simulink model "test_pmsm_inverter"  (R2026b)
settings: Solver=ode23tb  StopTime=tb.t_stop
undefined symbols (not defined in the file or in its folder): mach, tb
libraries: fl_lib x6, nesl_utility x3, permanent_magnet_synchronous_machine x1, pmsm_inverter_dqctrl x1
settings Model: Creator=pwr-control  LastModifiedBy=dbagn
settings SolverCC: ZeroCrossAlgorithm=Adaptive  ZeroCrossControl=EnableAll
settings DataIOCC: SaveOutput=off
settings SimscapeCC: SimscapeLogType=all  SimscapeNominalValues="[{\"value\":\"1\",\"unit\":\"A\"},{\"value\":\"1\",\"unit\":\"bar\"},{\"value\":\"1\",\"unit\":\"cm^2\"},{\"value\":\"1\",\"unit\":\"cm^3/s\"},{\"value\":\"1\",\"unit\":\"kJ/kg\"},{\"value\":\"1\",\"unit\":\"kW\"},{\"value\":\"1\",\"unit\":\"l\"},{\"value\":\"1\",\"unit\":\"N\"},{\"value\":\"1\",\"unit\":\"N*m\"},{\"value\":\"1\",\"unit\":\"V\"},{\"value\":\"0.001\",\"unit\":\"Wb\"}]"  SimscapeUseEnergyAccounting=off

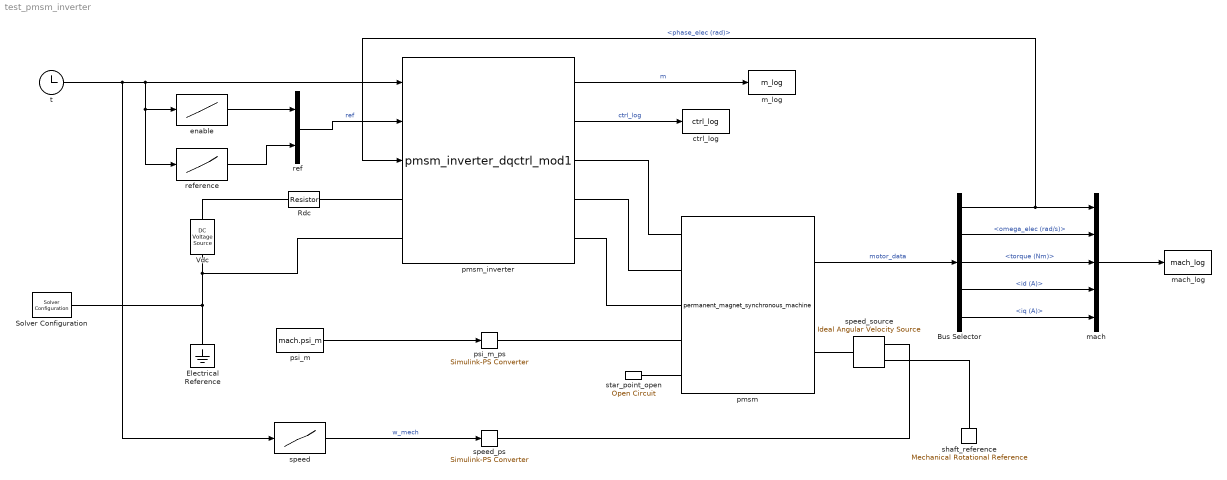
== system test_pmsm_inverter ==
  Bus Selector : BusSelector  OutputSignals=phase_elec (rad),omega_elec (rad/s),torque (Nm),id (A),iq (A)
  Electrical Reference : fl_lib/Electrical/Electrical Elements/Electrical Reference
  Rdc : fl_lib/Electrical/Electrical Elements/Resistor  R=tb.Rdc Ohm  i_specify=off  i_priority=None  i=0 A  i_nominal_specify=off  i_nominal_value=1  i_nominal_unit=A  v_specify=off  v_priority=None  v=0 V  v_nominal_specify=off  v_nominal_value=1  v_nominal_unit=V
  Solver Configuration : nesl_utility/Solver Configuration  PhysicalDomain=network_engine_domain  SubClassName=solver  LeftPortType=input  RightPortType=generic  Tones=[]  Harmonics=[]  SimulateNoise=off  Profile=off  UseLocalSampling=off  EnableSwitchedLinearOptims=on  FrequencyDomain=off  UseCCode=off  RelTol=0.001  AbsTol=0.001  MinStep=1e-09  ToWorkspace=off  RevertToSquareIcSolve=off  NumHomotopyIterations=100  PhasorMode=off  PhasorModeNumHarmonics=1  ConsistencySolver=NEWTON_FTOL  CanonicalOrdering=UNORDERED  OptimizeIntermediates=UNOPTIMIZED  MulticoreSolverChoice=BACKWARD_EULER  IndexReductionMethod=DerivativeReplacement  DoDC=off  ResidualTolerance=1e-4  ConsistencyTolSource=GLOBAL  ConsistencyAbsTol=0.001  ConsistencyRelTol=0.001  ConsistencyTolFactor=0.001  UseLocalSolver=on  LocalSolverChoice=NE_BACKWARD_EULER_ADVANCER  ResolveIndetEquations=on  FunctionEvalNumThread=1  LocalSolverSampleTime=tb.tc  DoFixedCost=on  MaxNonlinIter=tb.nonlin_iter  MaxModeIter=tb.mode_iter  ComputeImpulses=off  ImpulseIterations=2  LinearAlgebra=auto  LinearAlgebraNumThread=0  EquationFormulation=NE_TIME_EF  DelaysMemoryBudget=1024  AutomaticFiltering=on  FilteringTimeConstant=0.001  PartitionStorageMethod=AS_NEEDED  PartitionMemoryBudget=1024  PartitionMethod=BALANCED  MultibodyUseLocalSolver=off  MultibodyLocalSolverChoice=ODE1  MultibodyLocalSolverSampleTime=0.001
  Vdc : fl_lib/Electrical/Electrical Sources/DC Voltage Source  v0=tb.Vdc V
  ctrl_log : ToWorkspace  VariableName=ctrl_log  SaveFormat=Timeseries  SampleTime=tb.ts_log
  enable : Lookup_n-D  NumberOfTableDimensions=1  BreakpointsForDimension1=tb.prof.t  Table=tb.prof.enable  InternalRulePriority=Speed  RndMeth=Simplest
  m_log : ToWorkspace  VariableName=m_log  SaveFormat=Timeseries  SampleTime=tb.ts_log
  mach : Mux  Inputs=5
  mach_log : ToWorkspace  VariableName=mach_log  SaveFormat=Timeseries  SampleTime=tb.ts_log
  pmsm : permanent_magnet_synchronous_machine/permanent_magnet_synchronous_machine  pp=mach.poles  psi_m=mach.psi_m  Lmu=mach.Lmu  La=(mach.Ld + mach.Lq)/3  Lb=(mach.Lq - mach.Ld)/3  Rs=mach.Rs  Jm=mach.J  b_linear=0  b_quadratic=0  h5_percent=0  h7_percent=0  psi_r_u_init=mach.psi_m*cos(tb.theta0)  psi_r_v_init=mach.psi_m*cos(tb.theta0 - 2*pi/3)  psi_r_w_init=mach.psi_m*cos(tb.theta0 + 2*pi/3)  omega_init=tb.omega_e0  phase_init=tb.theta0  angle_error=0
  pmsm_inverter : pmsm_inverter_dqctrl/pmsm_inverter_dqctrl_mod1  p=p_inv
  psi_m : Constant  Value=mach.psi_m
  psi_m_ps : nesl_utility/Simulink-PS Converter  PhysicalDomain=network_engine_domain  SubClassName=ps_input  LeftPortType=input  RightPortType=output  PseudoPeriodic=off  Frequencies=[]  NoiseDistribution=none  NoiseParameters=[]  Unit=V*s  AffineConversion=off  FilteringAndDerivatives=provide  SimscapeFilterOrder=1  InputFilterTimeConstant=0.001  UdotUserProvided=0
  ref : Mux  Inputs=2
  reference : Lookup_n-D  NumberOfTableDimensions=1  BreakpointsForDimension1=tb.prof.t  Table=tb.prof.ref  InternalRulePriority=Speed  RndMeth=Simplest
  shaft_reference : fl_lib/Mechanical/Rotational Elements/Mechanical Rotational Reference
  speed : Lookup_n-D  NumberOfTableDimensions=1  BreakpointsForDimension1=tb.prof.t  Table=tb.prof.w_mech  InternalRulePriority=Speed  RndMeth=Simplest
  speed_ps : nesl_utility/Simulink-PS Converter  PhysicalDomain=network_engine_domain  SubClassName=ps_input  LeftPortType=input  RightPortType=output  PseudoPeriodic=off  Frequencies=[]  NoiseDistribution=none  NoiseParameters=[]  Unit=rad/s  AffineConversion=off  FilteringAndDerivatives=filter  SimscapeFilterOrder=1  InputFilterTimeConstant=tb.w_tau  UdotUserProvided=0
  speed_source : fl_lib/Mechanical/Mechanical Sources/Ideal Angular Velocity Source
  star_point_open : fl_lib/Electrical/Electrical Elements/Open Circuit  v_specify=off  v_priority=None  v=0 V  v_nominal_specify=off  v_nominal_value=1  v_nominal_unit=V
  t : Clock
  wires:
  t/1 -> enable/1, reference/1, pmsm_inverter/1, speed/1
  Bus Selector/2 -> mach/2  "<omega_elec (rad/s)>"
  pmsm/1 -> Bus Selector/1  "motor_data"
  enable/1 -> ref/1
  reference/1 -> ref/2
  pmsm_inverter/2 -> ctrl_log/1  "ctrl_log"
  ref/1 -> pmsm_inverter/2  "ref"
  psi_m/1 -> psi_m_ps/1
  speed/1 -> speed_ps/1  "w_mech"
  pmsm_inverter/1 -> m_log/1  "m"
  Bus Selector/5 -> mach/5  "<iq (A)>"
  Bus Selector/1 -> mach/1, pmsm_inverter/3  "<phase_elec (rad)>"
  Bus Selector/3 -> mach/3  "<torque (Nm)>"
  Bus Selector/4 -> mach/4  "<id (A)>"
  mach/1 -> mach_log/1
  connections:
  speed_ps/RConn1 -- speed_source/RConn1
  Solver Configuration/RConn1 -- pmsm_inverter/LConn2 -- Vdc/RConn1 -- Electrical Reference/LConn1
  Rdc/RConn1 -- pmsm_inverter/LConn1
  pmsm_inverter/RConn3 -- pmsm/LConn3
  pmsm_inverter/RConn1 -- pmsm/LConn1
  Vdc/LConn1 -- Rdc/LConn1
  pmsm_inverter/RConn2 -- pmsm/LConn2
  psi_m_ps/RConn1 -- pmsm/LConn4
  star_point_open/LConn1 -- pmsm/LConn5
  pmsm/RConn1 -- speed_source/LConn1
  speed_source/RConn2 -- shaft_reference/LConn1
